simulink model "controller"  (R2025b)
settings: Solver=FixedStepAuto  StartTime=0.0  StopTime=2500  FixedStep=0.1  RelTol=1e-3
values from neighbouring files (symbols this model uses):
  fn1_fit = fn_fit(:,1)    [Experimental_project_latest.m]
  fn2_fit = fn_fit(:,2)    [Experimental_project_latest.m]
  max_f1_M = fn1_fit(1)    [Experimental_project_latest.m]
  max_f2_M = fn2_fit(1)    [Experimental_project_latest.m]
  P_inv1_A = polyfit(fn1_fit(min_idx1:end), currents(min_idx1:end), 3)    [Experimental_project_latest.m]
  P_inv1_M = polyfit(fn1_fit(1:min_idx1), currents(1:min_idx1), 2)    [Experimental_project_latest.m]
  P_inv2_A = polyfit(fn2_fit(min_idx2:end), currents(min_idx2:end), 3)    [Experimental_project_latest.m]
  P_inv2_M = polyfit(fn2_fit(1:min_idx2), currents(1:min_idx2), 2)    [Experimental_project_latest.m]
libraries: simulink x1
settings Model: Creator=asus  LastModifiedBy=asus

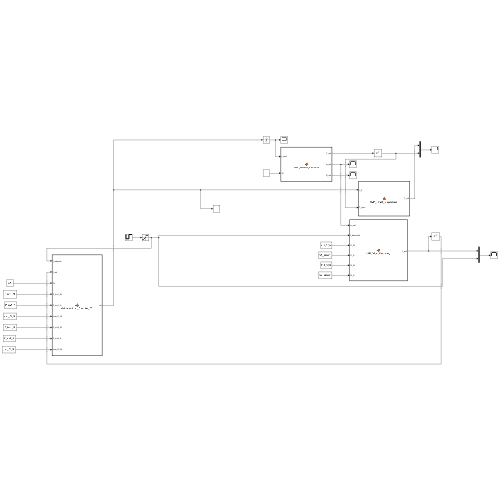
[thumbnail: Simulink's stored preview of the top-level diagram]
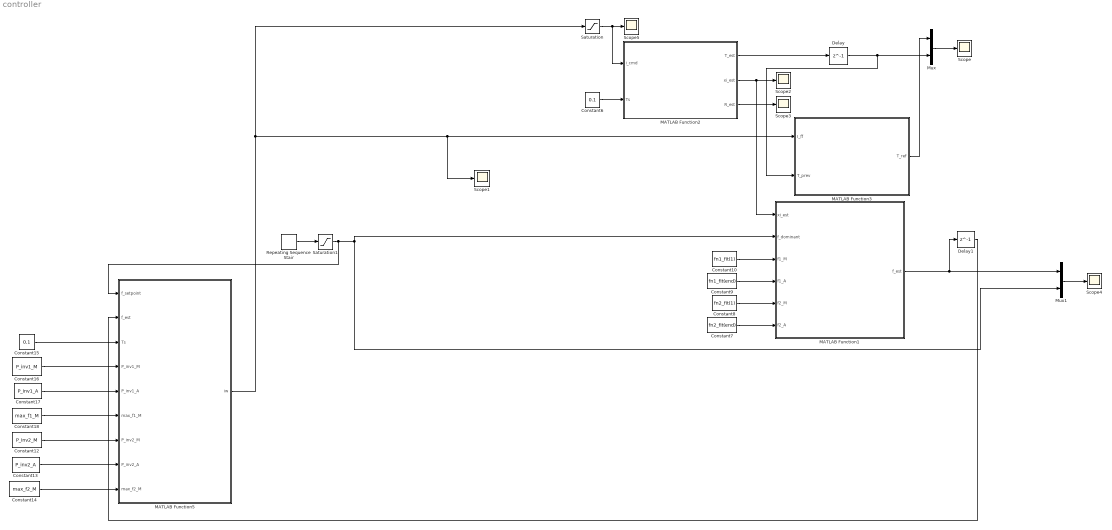
== system controller ==
  Constant10 : Constant  Value=fn1_fit(1)
  Constant12 : Constant  Value=P_inv2_M
  Constant13 : Constant  Value=P_inv2_A
  Constant14 : Constant  Value=max_f2_M
  Constant15 : Constant  Value=0.1
  Constant16 : Constant  Value=P_inv1_M
  Constant17 : Constant  Value=P_inv1_A
  Constant18 : Constant  Value=max_f1_M
  Constant6 : Constant  Value=0.1
  Constant7 : Constant  Value=fn2_fit(end)
  Constant8 : Constant  Value=fn2_fit(1)
  Constant9 : Constant  Value=fn1_fit(end)
  Delay : Delay  DelayLength=1  InitialCondition=20  SampleTime=0.1
  Delay1 : Delay  DelayLength=1  InitialCondition=fn2_fit(1)  SampleTime=0.1
  MATLAB Function1 : MATLAB Function  TreatAsAtomicUnit=on
  MATLAB Function2 : MATLAB Function  TreatAsAtomicUnit=on
  MATLAB Function3 : MATLAB Function  TreatAsAtomicUnit=on
  MATLAB Function5 : MATLAB Function  TreatAsAtomicUnit=on
  Mux : Mux  Inputs=2
  Mux1 : Mux  Inputs=2
  Repeating Sequence Stair : simulink/Sources/Repeating Sequence Stair  OutValues=[18.9 23.9].'  tsamp=250  OutMin=[]  OutMax=[]  OutDataTypeStr=double  OutputDataTypeScalingMode=double  OutDataType=fixdt(0,8)  ConRadixGroup=Best Precision: Vector-wise  OutScaling=2^-12
  Saturation : Saturate  UpperLimit=9.5  LowerLimit=0
  Saturation1 : Saturate  UpperLimit=26  LowerLimit=16
  Scope{,1..5} (6 alike) : Scope
      Scope settings: ActiveDisplayYMinimum=-263.90577941937261  ActiveDisplayYMaximum=171.64626163567155
      Scope1 settings: ActiveDisplayYMinimum=-1.1874999999999998  ActiveDisplayYMaximum=10.6875
      Scope2 settings: ActiveDisplayYMinimum=-6.2401863776620221  ActiveDisplayYMaximum=6.5348107473374935  DataLoggingVariableName=ScopeData2
      Scope3 settings: ActiveDisplayYMinimum=0.045200003838098295  ActiveDisplayYMaximum=0.051566201561774105  DataLoggingVariableName=ScopeData3
      Scope4 settings: ActiveDisplayYMinimum=0.88658588868715071  ActiveDisplayYMaximum=34.608656177278561  DataLoggingVariableName=ScopeData4
      Scope5 settings: ActiveDisplayYMinimum=-1.1874999999999998  ActiveDisplayYMaximum=10.6875  DataLoggingVariableName=ScopeData5
  wires:
  Mux1/1 -> Scope4/1
  Saturation1/1 -> MATLAB Function5/1(f_setpoint), Mux1/2, MATLAB Function1/2(f_dominant)
  Repeating Sequence Stair/1 -> Saturation1/1
  Saturation/1 -> MATLAB Function2/1(i_cmd), Scope5/1
  Constant6/1 -> MATLAB Function2/2(Ts)
  MATLAB Function2/1(T_est) -> Delay/1
  MATLAB Function2/2(xi_est) -> Scope2/1, MATLAB Function1/1(xi_est)
  MATLAB Function2/3(R_est) -> Scope3/1
  Constant10/1 -> MATLAB Function1/3(f1_M)
  MATLAB Function1/1(f_est) -> Mux1/1, Delay1/1
  Constant9/1 -> MATLAB Function1/4(f1_A)
  MATLAB Function3/1(T_ref) -> Mux/1
  Constant8/1 -> MATLAB Function1/5(f2_M)
  Constant7/1 -> MATLAB Function1/6(f2_A)
  Delay/1 -> MATLAB Function3/2(T_prev), Mux/2
  Mux/1 -> Scope/1
  Delay1/1 -> MATLAB Function5/2(f_est)
  Constant14/1 -> MATLAB Function5/9(max_f2_M)
  Constant13/1 -> MATLAB Function5/8(P_inv2_A)
  Constant12/1 -> MATLAB Function5/7(P_inv2_M)
  Constant15/1 -> MATLAB Function5/3(Ts)
  Constant17/1 -> MATLAB Function5/5(P_inv1_A)
  Constant16/1 -> MATLAB Function5/4(P_inv1_M)
  Constant18/1 -> MATLAB Function5/6(max_f1_M)
  MATLAB Function5/1(iw) -> Scope1/1, MATLAB Function3/1(I_ff), Saturation/1

== matlab function controller/MATLAB Function1 ==
  settings: updateMethod=DISCRETE
  data: xi_est input; f_dominant input; f_est output; f1_M input; f1_A input; f2_M input; f2_A input
function f_est = SMA_Xi_to_Frequency(xi_est, f_dominant, f1_M, f1_A, f2_M, f2_A)
% xi_est      : current phase fraction estimate (1 = martensite, 0 = austenite)
% f_dominant  : your frequency SETPOINT (used only to pick which mode band
%               is currently being targeted, same logic as your
%               ATMD_Supervisory_Controller)
% f1_M, f1_A  : mode 1 endpoint frequencies [Hz], fully martensite / fully austenite
% f2_M, f2_A  : mode 2 endpoint frequencies [Hz], fully martensite / fully austenite

f_est = 0;

if f_dominant >= 16 && f_dominant <= 40
    r = f1_A / f1_M;
    ratio_sq = xi_est + (1 - xi_est)*r^2;
    if ratio_sq < 0, ratio_sq = 0; end
    f_est = f1_M * sqrt(ratio_sq);

elseif f_dominant >= 260 && f_dominant <= 350
    r = f2_A / f2_M;
    ratio_sq = xi_est + (1 - xi_est)*r^2;
    if ratio_sq < 0, ratio_sq = 0; end
    f_est = f2_M * sqrt(ratio_sq);
end
end

== matlab function controller/MATLAB Function2 ==
  settings: updateMethod=DISCRETE
  data: i_cmd input; Ts input; T_est output; xi_est output; R_est output
function [T_est, xi_est, R_est] = SMA_Thermal_Observer(i_cmd, Ts)

Aext = pi*0.004*0.140*2;  h = 15;  m_mass = 0.0099;  cp = 500;  T0 = 20;
rho_a = 100e-8; rho_m = 90e-8; Ltot = 0.280; Area = pi*(0.002^2-0.0015^2);
As = 55.0; Af = 65.0; Ms = 40.0; Mf = 28.5;

persistent T xi_prev R_prev initialized
if isempty(initialized)
    T = T0; xi_prev = 1; R_prev = rho_m*Ltot/Area; initialized = true;
end

% ---- OUTPUT the state as it stood BEFORE this call's input is applied ----
T_est  = T;
xi_est = xi_prev;
R_est  = R_prev;

% ---- Now update state for the NEXT call, using this call's i_cmd ----
xi_heat = xi_branch_heating(T, As, Af);
xi_cool = xi_branch_cooling(T, Ms, Mf);
if xi_heat <= xi_prev
    xi = xi_heat;
else
    xi = xi_cool;
end

rho  = rho_a + xi*(rho_m - rho_a);
R    = rho*Ltot/Area;
dTdt = (R*i_cmd^2 - Aext*h*(T - T0)) / (m_mass*cp);
T    = T + Ts*dTdt;

xi_prev = xi;
R_prev  = R;
end

function xi = xi_branch_heating(T, As, Af)
if T <= As, xi = 1; elseif T < Af, xi = (Af-T)/(Af-As); else, xi = 0; end
end
function xi = xi_branch_cooling(T, Ms, Mf)
if T >= Ms, xi = 0; elseif T > Mf, xi = (Ms-T)/(Ms-Mf); else, xi = 1; end
end

== matlab function controller/MATLAB Function3 ==
  data: I_ff input; T_ref output; T_prev input
function T_ref = SMA_Target_Temperature(I_ff, T_prev)
% T_prev: pass in the observer's own T_est (delayed) so this function knows
% whether the system is currently above or below where heating/cooling splits.
Aext = pi*0.004*0.140*2;  h = 15;  T0 = 20;
rho_a = 100e-8; rho_m = 90e-8; Ltot = 0.280; Area = pi*(0.002^2-0.0015^2);
As = 55.0; Af = 65.0; Ms = 40.0; Mf = 28.5;

T = T_prev;   % start iteration from current known state, not always T0
for k = 1:15
    if I_ff > 0
        xi = xi_branch_heating(T, As, Af);
    else
        xi = xi_branch_cooling(T, Ms, Mf);
    end
    rho = rho_a + xi*(rho_m - rho_a);
    R   = rho*Ltot/Area;
    T   = T0 + (R*I_ff^2)/(Aext*h);
end
T_ref = T;
end

function xi = xi_branch_heating(T, As, Af)
if T <= As, xi = 1; elseif T < Af, xi = (Af-T)/(Af-As); else, xi = 0; end
end
function xi = xi_branch_cooling(T, Ms, Mf)
if T >= Ms, xi = 0; elseif T > Mf, xi = (Ms-T)/(Ms-Mf); else, xi = 1; end
end

== matlab function controller/MATLAB Function5 ==
  data: f_setpoint input; iw output; f_est input; Ts input; P_inv1_M input; P_inv1_A input; max_f1_M input; P_inv2_M input; P_inv2_A input; max_f2_M input
function iw = GainScheduled_Controller_FF(f_setpoint, f_est, Ts, ...
    P_inv1_M, P_inv1_A, max_f1_M, P_inv2_M, P_inv2_A, max_f2_M)

tol = 0.3;
kp_heat = 0.05;  ki_heat = 0.01;
kp_cool = 0.02;  ki_cool = 0.005;
i_min = 0;  i_max = 9.5;

% ---- Feedforward: pick mode band first, then heating/cooling branch ----
if f_setpoint >= 16 && f_setpoint <= 40
    if f_setpoint <= max_f1_M
        I_ff = polyval(P_inv1_M, f_setpoint);
    else
        I_ff = polyval(P_inv1_A, f_setpoint);
    end
elseif f_setpoint >= 260 && f_setpoint <= 350
    if f_setpoint <= max_f2_M
        I_ff = polyval(P_inv2_M, f_setpoint);
    else
        I_ff = polyval(P_inv2_A, f_setpoint);
    end
else
    I_ff = 0;   % setpoint outside any known band -- flag this rather than guess
end
I_ff = min(max(I_ff, i_min), i_max);

% ---- rest unchanged from before ----
persistent integ iw_last initialized
if isempty(initialized)
    integ = 0; iw_last = I_ff; initialized = true;
end

e = f_setpoint - f_est;
if e > tol
    iw_unclamped = I_ff + kp_heat*e + ki_heat*integ;
elseif e < -tol
    iw_unclamped = I_ff + kp_cool*e + ki_cool*integ;
else
    iw_unclamped = iw_last;
end

iw = min(max(iw_unclamped, i_min), i_max);
if abs(e) > tol
    if iw_unclamped == iw || (iw_unclamped > i_max && e < 0) || (iw_unclamped < i_min && e > 0)
        integ = integ + e*Ts;
    end
end
iw_last = iw;
end
